simulink model "BallBeam1"  (R2016b)
settings: Solver=ode45  StartTime=0.0  StopTime=5  RelTol=1e-3
InitFcn:
  | init
values from neighbouring files (symbols this model uses):
  A = [0 1 0 0 ... (first row only)    [Tarsgo.m]
  B = [0 ... (first row only)    [Tarsgo.m]
  g = 9.8    [Tarsgo.m]    (also in nonlinear_model.m; nonlinear_model1.m)
  J = 2e-3    (= 0.002)    [Tarsgo.m]    (also in nonlinear_model.m; nonlinear_model1.m)
  Jr = 1e-5    (= 1e-05)    [Tarsgo.m]    (also in nonlinear_model.m; nonlinear_model1.m)
  m = 0.11    [Tarsgo.m]    (also in nonlinear_model.m; nonlinear_model1.m)
  R = 1    [Tarsgo.m]    (also in nonlinear_model.m = 0.015; nonlinear_model1.m = 0.015)
  x0 = [0.5 0.2 1 0.3]    [Tarsgo.m]
settings Model: Creator=Mojtaba  LastModifiedBy=Mojtaba

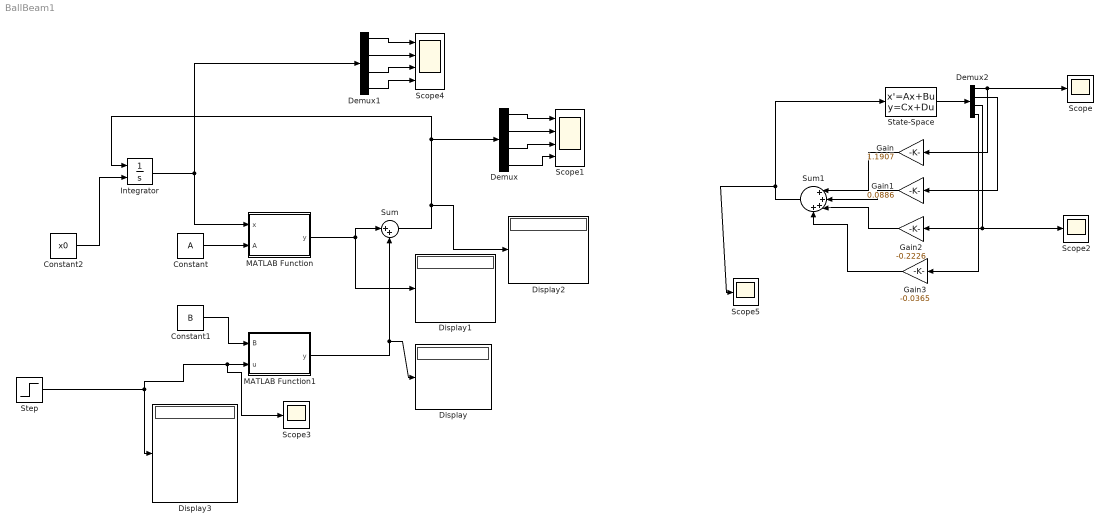
== system BallBeam1 ==
  Constant : Constant  Value=A
  Constant1 : Constant  Value=B
  Constant2 : Constant  Value=x0
  Demux : Demux
  Demux1 : Demux
  Demux2 : Demux
  Display{,1..3} (4 alike) : Display
  Gain : Gain  Gain=1.1907
  Gain1 : Gain  Gain=0.0886
  Gain2 : Gain  Gain=-0.2226
  Gain3 : Gain  Gain=-0.0365
  Integrator : Integrator  InitialConditionSource=external  InitialCondition=x0
  MATLAB Function : MATLAB Function  TreatAsAtomicUnit=on
  MATLAB Function1 : MATLAB Function  TreatAsAtomicUnit=on
  Scope{,2..3,5} (4 alike) : Scope
  Scope1 : Scope  NumInputPorts=4
  Scope4 : Scope  NumInputPorts=4
  State-Space : StateSpace  A=[0 1 0 0;(-Jr/R*m*g)/(m*(J+Jr)+J*Jr/R^2) 0 -(J+Jr)*m*g/(m*(J+Jr)+J*Jr/R^2) 0;0 0 0 1; -(m+Jr/R^2)*m*g/(m*(J+Jr)+J*Jr/R^2) 0 -Jr/R*m*g/(m*(J+Jr)+J*Jr/R^2) 0]  B=[0;Jr/R/(m*(J+Jr)+J*Jr/R^2);0;(m+Jr/R^2)/(m*(J+Jr)+J*Jr/R^2)]  C=[1 0 0 0;0 1 0 0;0 0 1 0;0 0 0 1]  D=[0; 0; 0; 0]  X0=[.5 0.2 1 .3]
  Step : Step  Time=0.01  After=100  SampleTime=0
  Sum : Sum  Inputs=|++
  Sum1 : Sum  Inputs=|++++
  wires:
  MATLAB Function/1(y) -> Sum/1, Display1/1
  Sum/1 -> Display2/1, Demux/1, Integrator/1
  MATLAB Function1/1(y) -> Display/1, Sum/2
  Constant/1 -> MATLAB Function/2(A)
  Constant1/1 -> MATLAB Function1/1(B)
  Constant2/1 -> Integrator/2
  Demux/1 -> Scope1/1
  Demux/2 -> Scope1/2
  Demux/3 -> Scope1/3
  Demux/4 -> Scope1/4
  Demux1/1 -> Scope4/1
  Demux1/2 -> Scope4/2
  Demux1/3 -> Scope4/3
  Demux1/4 -> Scope4/4
  Step/1 -> Scope3/1, MATLAB Function1/2(u), Display3/1
  Integrator/1 -> MATLAB Function/1(x), Demux1/1
  State-Space/1 -> Demux2/1
  Demux2/1 -> Gain/1, Scope/1
  Demux2/2 -> Gain1/1
  Demux2/3 -> Gain2/1, Scope2/1
  Demux2/4 -> Gain3/1
  Gain/1 -> Sum1/1
  Gain1/1 -> Sum1/2
  Gain2/1 -> Sum1/3
  Gain3/1 -> Sum1/4
  Sum1/1 -> State-Space/1, Scope5/1

== matlab function BallBeam1/MATLAB Function1 ==
  data: B input; u input; y output
function y = fcn(B,u)
y =B*u;
end

== matlab function BallBeam1/MATLAB Function ==
  data: x input; A input; y output
function y = fcn(x,A)
y =A*x;
end
